simulink model "ackerman_ROS2_controller"  (R2025a)
settings: Solver=FixedStepDiscrete  StopTime=200  FixedStep=0.05  EnableMultiTasking=on
model workspace (MAT data in the model file):
  SL_ROS_VariableLengthArrays_MaxSizes.CommonInfo.ArrayTruncateAction = 'EmitWarning'
  SL_ROS_VariableLengthArrays_MaxSizes.MsgTypeMap = containers.Map
  SL_ROS_VariableLengthArrays_MaxSizes.MsgTypeMap.serialization.keys = {'sensor_msgs/LaserScan'}
  SL_ROS_VariableLengthArrays_MaxSizes.MsgTypeMap.serialization.values{1}(1).PropertyName = 'intensities'
  SL_ROS_VariableLengthArrays_MaxSizes.MsgTypeMap.serialization.values{1}(1).DataType = 'single'
  SL_ROS_VariableLengthArrays_MaxSizes.MsgTypeMap.serialization.values{1}(1).MaxLength = 90
  SL_ROS_VariableLengthArrays_MaxSizes.MsgTypeMap.serialization.values{1}(2).PropertyName = 'ranges'
  SL_ROS_VariableLengthArrays_MaxSizes.MsgTypeMap.serialization.values{1}(2).DataType = 'single'
  SL_ROS_VariableLengthArrays_MaxSizes.MsgTypeMap.serialization.values{1}(2).MaxLength = 90
  SL_ROS_VariableLengthArrays_MaxSizes.MsgTypeMap.serialization.uniformity = 0
  SL_ROS_VariableLengthArrays_MaxSizes.MsgTypeMap.serialization.keyType = 'char'
  SL_ROS_VariableLengthArrays_MaxSizes.MsgTypeMap.serialization.valueType = 'any'
undefined symbols (not defined in the file or in its folder): angular, linear
libraries: ros2lib x13, fuzblock x1, robotcorelib x1
settings Model: Creator=pizarro  LastModifiedBy=rodrigo.gutierrez
settings SolverCC: AlgebraicLoopSolver=TrustRegion
settings OptimizationCC: ReuseModelBlockBuffer=off
settings DebuggingCC: UnconnectedInputMsg=warning  UnconnectedOutputMsg=warning  UnconnectedLineMsg=warning
settings ModelReferenceCC: EnableRefExpFcnMdlSchedulingChecks=on
settings SFSimCC: SimGPUStackLimitPerThread=51200  SimGPUMallocThreshold=200  CustomCodeUndefinedFunction=UseInterfaceOnly
settings RTWCC: GPUStackLimitPerThread=51200  GPUMallocThreshold=200  GPUComputeCapability=3.5

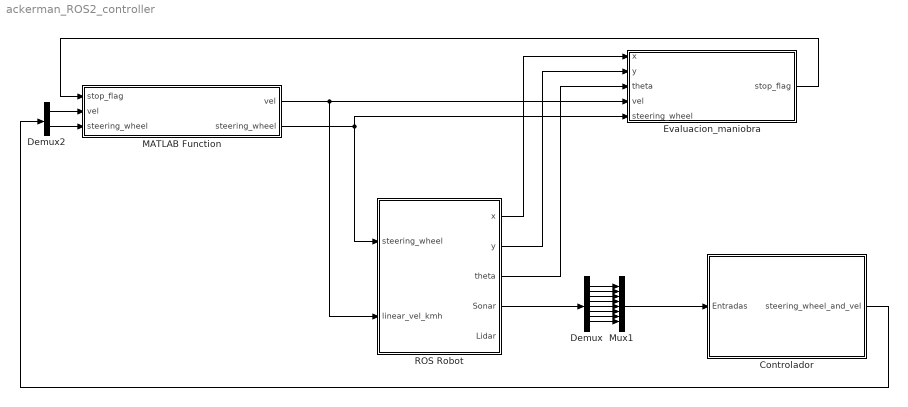
== system ackerman_ROS2_controller ==
  Controlador : Subsystem
  Demux : Demux  Outputs=8
  Demux2 : Demux  Outputs=2
  Evaluacion_maniobra : Subsystem
  MATLAB Function : MATLAB Function  TreatAsAtomicUnit=on
  Mux1 : Mux  Inputs=8
  ROS Robot : Subsystem
  wires:
  ROS Robot/1(x) -> Evaluacion_maniobra/1(x)
  ROS Robot/2(y) -> Evaluacion_maniobra/2(y)
  ROS Robot/3(theta) -> Evaluacion_maniobra/3(theta)
  Controlador/1(steering_wheel_and_vel) -> Demux2/1
  Evaluacion_maniobra/1(stop_flag) -> MATLAB Function/1(stop_flag)
  MATLAB Function/1(vel) -> ROS Robot/2(linear_vel_kmh), Evaluacion_maniobra/4(vel)
  MATLAB Function/2(steering_wheel) -> Evaluacion_maniobra/5(steering_wheel), ROS Robot/1(steering_wheel)
  Demux2/1 -> MATLAB Function/2("vel ")
  Demux2/2 -> MATLAB Function/3("steering_wheel ")
  Mux1/1 -> Controlador/1(Entradas)
  ROS Robot/4(Sonar) -> Demux/1
  Demux/1 -> Mux1/1
  Demux/2 -> Mux1/2
  Demux/3 -> Mux1/3
  Demux/4 -> Mux1/4
  Demux/5 -> Mux1/5
  Demux/6 -> Mux1/6
  Demux/7 -> Mux1/7
  Demux/8 -> Mux1/8

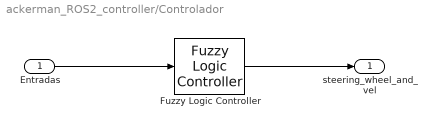
== system ackerman_ROS2_controller/Controlador ==
  Entradas : Inport
  Fuzzy Logic Controller : fuzblock/Fuzzy Logic  Controller  FIS='fuzzy_controller.fis'  OutputSampleNumber=1001  DataType=double  UseLookupTable=off  NumBreakpoints=10  FuzzifiedInputs=off  RuleFiringStrengths=off  RuleOutputs=off  AggregatedOutputs=off  SimulateUsing=Interpreted execution  OutOfRangeInputValueMessage=warning  NoRuleFiredMessage=warning  EmptyOutputFuzzySetMessage=warning
  steering_wheel_and_vel : Outport  VectorParamsAs1DForOutWhenUnconnected=off
  wires:
  Fuzzy Logic Controller/1 -> steering_wheel_and_vel/1
  Entradas/1 -> Fuzzy Logic Controller/1

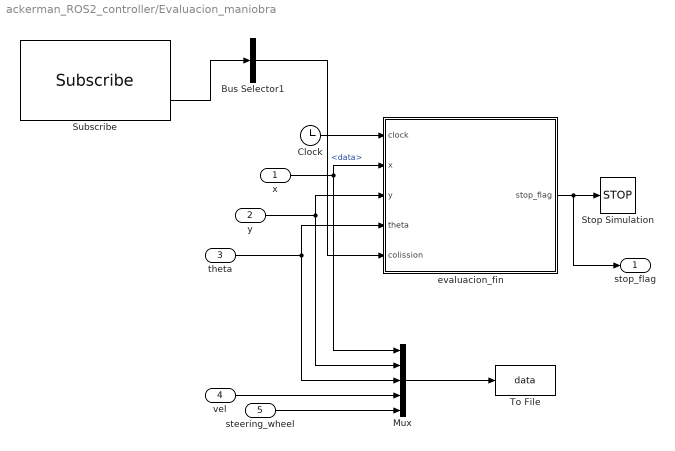
== system ackerman_ROS2_controller/Evaluacion_maniobra ==
  x : Inport
  y : Inport  Port=2
  theta : Inport  Port=3
  vel : Inport  Port=4
  steering_wheel : Inport  Port=5
  Bus Selector1 : BusSelector  OutputSignals=data
  Clock : Clock
  Mux : Mux  Inputs=5
  Stop Simulation : Stop
  Subscribe : ros2lib/Subscribe  topicSource=Select from ROS network  topic=/r0/collision  messageType=std_msgs/Bool  SubscriberMode=At sample time  sampleTime=-1  CallbackGroupType=Default  CallbackGroupName=callback_group_1  QOSHistory=Keep last  QOSDepth=10  QOSReliability=Reliable  QOSDurability=Volatile  QOSDeadline=Inf  QOSLifespan=Inf  QOSLiveliness=Automatic  QOSLeaseDuration=Inf  QOSAvoidROSNamespaceConventions=off
  To File : ToFile  Filename=data  MatrixName=data
  evaluacion_fin : MATLAB Function  TreatAsAtomicUnit=on
  stop_flag : Outport
  wires:
  theta/1 -> Mux/3, evaluacion_fin/4(theta)
  Clock/1 -> evaluacion_fin/1(clock)
  y/1 -> Mux/2, evaluacion_fin/3(y)
  evaluacion_fin/1(stop_flag) -> stop_flag/1, Stop Simulation/1
  Mux/1 -> To File/1
  x/1 -> Mux/1, evaluacion_fin/2(x)
  vel/1 -> Mux/4
  steering_wheel/1 -> Mux/5
  Subscribe/2 -> Bus Selector1/1
  Bus Selector1/1 -> evaluacion_fin/5(colission)  "<data>"

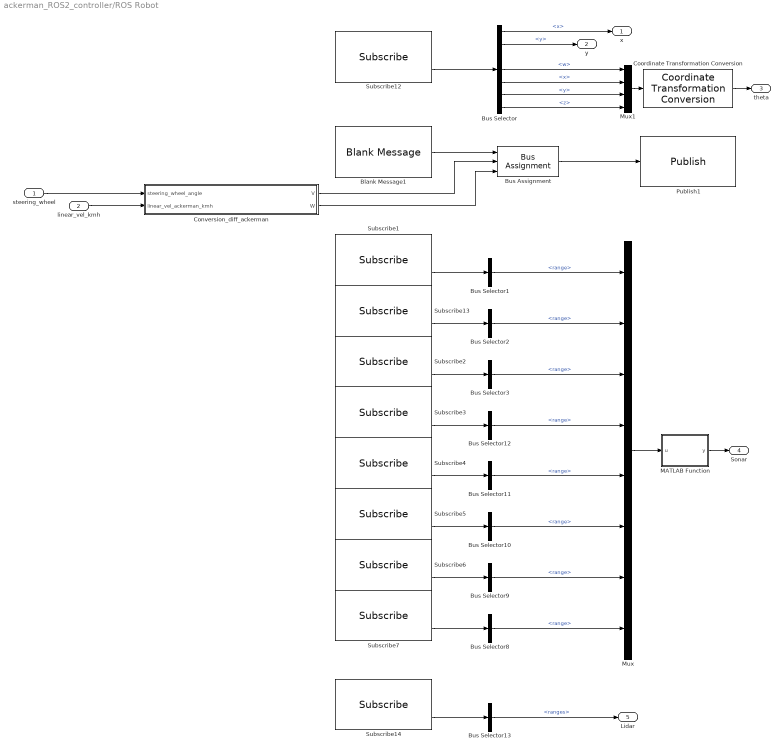
== system ackerman_ROS2_controller/ROS Robot ==
  steering_wheel : Inport
  linear_vel_kmh : Inport  Port=2
  Blank Message1 : ros2lib/Blank Message  messageClass=Message  entityType=geometry_msgs/Twist  messageType=geometry_msgs/Twist  SampleTime=inf
  Bus Assignment : BusAssignment  AssignedSignals=linear.x,angular.z
  Bus Selector : BusSelector  OutputSignals=pose.pose.position.x,pose.pose.position.y,pose.pose.position.z,pose.pose.orientation.w,pose.pose.orientation.x,pose.pose.orientation.y,pose.pose.orientation.z
  Bus Selector{1..3,8..12} (8 alike) : BusSelector  OutputSignals=range
  Bus Selector13 : BusSelector  OutputSignals=ranges
  Conversion_diff_ackerman : MATLAB Function  TreatAsAtomicUnit=on
  Coordinate Transformation Conversion : robotcorelib/Coordinate Transformation Conversion  InputRepresentation=Quaternion  InputEulerSequence=ZYX  ShowTrVecInputPort=on  OutputRepresentation=Euler Angles  OutputEulerSequence=ZYX  ShowTrVecOutputPort=on  SimulateUsing=Interpreted execution
  MATLAB Function : MATLAB Function  TreatAsAtomicUnit=on
  Mux : Mux  Inputs=8
  Mux1 : Mux
  Publish1 : ros2lib/Publish  topicSource=Select from ROS network  topic=/r0/cmd_vel  messageType=geometry_msgs/Twist  QOSHistory=Keep last  QOSDepth=10  QOSReliability=Reliable  QOSDurability=Volatile  QOSDeadline=Inf  QOSLifespan=Inf  QOSLiveliness=Automatic  QOSLeaseDuration=Inf  QOSAvoidROSNamespaceConventions=off
  Subscribe1 : ros2lib/Subscribe  topicSource=Select from ROS network  topic=/r0/sonar0  messageType=sensor_msgs/Range  SubscriberMode=At sample time  sampleTime=-1  CallbackGroupType=Default  CallbackGroupName=callback_group_1  QOSHistory=Keep last  QOSDepth=10  QOSReliability=Reliable  QOSDurability=Volatile  QOSDeadline=Inf  QOSLifespan=Inf  QOSLiveliness=Automatic  QOSLeaseDuration=Inf  QOSAvoidROSNamespaceConventions=off
  Subscribe12 : ros2lib/Subscribe  topicSource=Select from ROS network  topic=/r0/odom  messageType=nav_msgs/Odometry  SubscriberMode=At sample time  sampleTime=-1  CallbackGroupType=Default  CallbackGroupName=callback_group_1  QOSHistory=Keep last  QOSDepth=10  QOSReliability=Reliable  QOSDurability=Volatile  QOSDeadline=Inf  QOSLifespan=Inf  QOSLiveliness=Automatic  QOSLeaseDuration=Inf  QOSAvoidROSNamespaceConventions=off
  Subscribe13 : ros2lib/Subscribe  topicSource=Select from ROS network  topic=/r0/sonar1  messageType=sensor_msgs/Range  SubscriberMode=At sample time  sampleTime=-1  CallbackGroupType=Default  CallbackGroupName=callback_group_1  QOSHistory=Keep last  QOSDepth=10  QOSReliability=Reliable  QOSDurability=Volatile  QOSDeadline=Inf  QOSLifespan=Inf  QOSLiveliness=Automatic  QOSLeaseDuration=Inf  QOSAvoidROSNamespaceConventions=off
  Subscribe14 : ros2lib/Subscribe  topicSource=Select from ROS network  topic=/r0/scan  messageType=sensor_msgs/LaserScan  SubscriberMode=At sample time  sampleTime=-1  CallbackGroupType=Default  CallbackGroupName=callback_group_1  QOSHistory=Keep last  QOSDepth=10  QOSReliability=Reliable  QOSDurability=Volatile  QOSDeadline=Inf  QOSLifespan=Inf  QOSLiveliness=Automatic  QOSLeaseDuration=Inf  QOSAvoidROSNamespaceConventions=off
  Subscribe2 : ros2lib/Subscribe  topicSource=Select from ROS network  topic=/r0/sonar2  messageType=sensor_msgs/Range  SubscriberMode=At sample time  sampleTime=-1  CallbackGroupType=Default  CallbackGroupName=callback_group_1  QOSHistory=Keep last  QOSDepth=10  QOSReliability=Reliable  QOSDurability=Volatile  QOSDeadline=Inf  QOSLifespan=Inf  QOSLiveliness=Automatic  QOSLeaseDuration=Inf  QOSAvoidROSNamespaceConventions=off
  Subscribe3 : ros2lib/Subscribe  topicSource=Select from ROS network  topic=/r0/sonar3  messageType=sensor_msgs/Range  SubscriberMode=At sample time  sampleTime=-1  CallbackGroupType=Default  CallbackGroupName=callback_group_1  QOSHistory=Keep last  QOSDepth=10  QOSReliability=Reliable  QOSDurability=Volatile  QOSDeadline=Inf  QOSLifespan=Inf  QOSLiveliness=Automatic  QOSLeaseDuration=Inf  QOSAvoidROSNamespaceConventions=off
  Subscribe4 : ros2lib/Subscribe  topicSource=Select from ROS network  topic=/r0/sonar4  messageType=sensor_msgs/Range  SubscriberMode=At sample time  sampleTime=-1  CallbackGroupType=Default  CallbackGroupName=callback_group_1  QOSHistory=Keep last  QOSDepth=10  QOSReliability=Reliable  QOSDurability=Volatile  QOSDeadline=Inf  QOSLifespan=Inf  QOSLiveliness=Automatic  QOSLeaseDuration=Inf  QOSAvoidROSNamespaceConventions=off
  Subscribe5 : ros2lib/Subscribe  topicSource=Select from ROS network  topic=/r0/sonar5  messageType=sensor_msgs/Range  SubscriberMode=At sample time  sampleTime=-1  CallbackGroupType=Default  CallbackGroupName=callback_group_1  QOSHistory=Keep last  QOSDepth=10  QOSReliability=Reliable  QOSDurability=Volatile  QOSDeadline=Inf  QOSLifespan=Inf  QOSLiveliness=Automatic  QOSLeaseDuration=Inf  QOSAvoidROSNamespaceConventions=off
  Subscribe6 : ros2lib/Subscribe  topicSource=Select from ROS network  topic=/r0/sonar6  messageType=sensor_msgs/Range  SubscriberMode=At sample time  sampleTime=-1  CallbackGroupType=Default  CallbackGroupName=callback_group_1  QOSHistory=Keep last  QOSDepth=10  QOSReliability=Reliable  QOSDurability=Volatile  QOSDeadline=Inf  QOSLifespan=Inf  QOSLiveliness=Automatic  QOSLeaseDuration=Inf  QOSAvoidROSNamespaceConventions=off
  Subscribe7 : ros2lib/Subscribe  topicSource=Select from ROS network  topic=/r0/sonar7  messageType=sensor_msgs/Range  SubscriberMode=At sample time  sampleTime=-1  CallbackGroupType=Default  CallbackGroupName=callback_group_1  QOSHistory=Keep last  QOSDepth=10  QOSReliability=Reliable  QOSDurability=Volatile  QOSDeadline=Inf  QOSLifespan=Inf  QOSLiveliness=Automatic  QOSLeaseDuration=Inf  QOSAvoidROSNamespaceConventions=off
  x : Outport  VectorParamsAs1DForOutWhenUnconnected=off
  y : Outport  Port=2  VectorParamsAs1DForOutWhenUnconnected=off
  theta : Outport  Port=3  VectorParamsAs1DForOutWhenUnconnected=off
  Sonar : Outport  Port=4  VectorParamsAs1DForOutWhenUnconnected=off
  Lidar : Outport  Port=5  VectorParamsAs1DForOutWhenUnconnected=off
  wires:
  Blank Message1/1 -> Bus Assignment/1
  Subscribe12/2 -> Bus Selector/1
  Bus Assignment/1 -> Publish1/1
  Subscribe1/2 -> Bus Selector1/1
  Conversion_diff_ackerman/1(V) -> Bus Assignment/2
  Conversion_diff_ackerman/2(W) -> Bus Assignment/3
  Subscribe13/2 -> Bus Selector2/1
  Subscribe2/2 -> Bus Selector3/1
  Subscribe4/2 -> Bus Selector11/1
  Subscribe3/2 -> Bus Selector12/1
  Subscribe5/2 -> Bus Selector10/1
  Subscribe6/2 -> Bus Selector9/1
  Bus Selector1/1 -> Mux/1  "<range>"
  Bus Selector2/1 -> Mux/2  "<range>"
  Bus Selector3/1 -> Mux/3  "<range>"
  Bus Selector12/1 -> Mux/4  "<range>"
  Bus Selector11/1 -> Mux/5  "<range>"
  Bus Selector10/1 -> Mux/6  "<range>"
  Bus Selector9/1 -> Mux/7  "<range>"
  Subscribe7/2 -> Bus Selector8/1
  Bus Selector8/1 -> Mux/8  "<range>"
  Mux1/1 -> Coordinate Transformation Conversion/1
  Coordinate Transformation Conversion/1 -> theta/1
  Mux/1 -> MATLAB Function/1(u)
  MATLAB Function/1(y) -> Sonar/1
  linear_vel_kmh/1 -> Conversion_diff_ackerman/2(linear_vel_ackerman_kmh)
  steering_wheel/1 -> Conversion_diff_ackerman/1(steering_wheel_angle)
  Subscribe14/2 -> Bus Selector13/1
  Bus Selector13/1 -> Lidar/1  "<ranges>"
  Bus Selector/1 -> x/1  "<x>"
  Bus Selector/2 -> y/1  "<y>"
  Bus Selector/4 -> Mux1/1  "<w>"
  Bus Selector/5 -> Mux1/2  "<x>"
  Bus Selector/6 -> Mux1/3  "<y>"
  Bus Selector/7 -> Mux1/4  "<z>"

== matlab function ackerman_ROS2_controller/ROS Robot/Conversion_diff_ackerman ==
  data: steering_wheel_angle input; V output; linear_vel_ackerman_kmh input; W output
function [V,W] = fcn(steering_wheel_angle, linear_vel_ackerman_kmh)
V = 0.0;
W = 0.0;
if ~isfinite(steering_wheel_angle) || ~isfinite(linear_vel_ackerman_kmh)
    return;
end
delta = min(45,max(-45,steering_wheel_angle))*pi/180;
V = min(50,max(0,linear_vel_ackerman_kmh))/3.6;
W = V*tan(delta)/0.3302;
end

== matlab function ackerman_ROS2_controller/ROS Robot/MATLAB Function ==
  data: u input; y output
function y = fcn(u)
y = u;
y(isinf(y) & y > 0) = 30;
y(~isfinite(y) | y < 0) = 0;
y = min(y,30);
end

== matlab function ackerman_ROS2_controller/MATLAB Function ==
  data: stop_flag input; vel output; vel input; steering_wheel input; steering_wheel output
function [vel, steering_wheel] = stop(stop_flag,vel,steering_wheel)
if stop_flag || ~isfinite(vel) || ~isfinite(steering_wheel)
    vel = 0.0;
    steering_wheel = 0.0;
else
    vel = min(50,max(0,vel));
    steering_wheel = min(45,max(-45,steering_wheel));
end
end

== matlab function ackerman_ROS2_controller/Evaluacion_maniobra/evaluacion_fin ==
  data: clock input; x input; y input; theta input; stop_flag output; colission input
function stop_flag = evaluacion_fin(clock, x, y, theta, colission)
persistent xAnterior vueltaIniciada
if isempty(xAnterior)
    xAnterior = 0;
    vueltaIniciada = false;
end
if clock == 0
    xAnterior = x;
    vueltaIniciada = false;
end
vueltaIniciada = vueltaIniciada || y > 0;
cruzaMeta = vueltaIniciada && xAnterior < 0 && x >= 0 && ...
    y > -14 && y < -10 && cos(theta(1)) > 0;
stop_flag = double(colission || cruzaMeta);
xAnterior = x;
end
